simulink model "reference_04_chain_loop_and_merge"  (R2026b)
settings: Solver=FixedStepDiscrete  StartTime=0  StopTime=0.5  FixedStep=0.01  RelTol=1e-10  AbsTol=1e-12
settings Model: Creator=Fasih  LastModifiedBy=Fasih
settings DataIOCC: SaveOutput=off

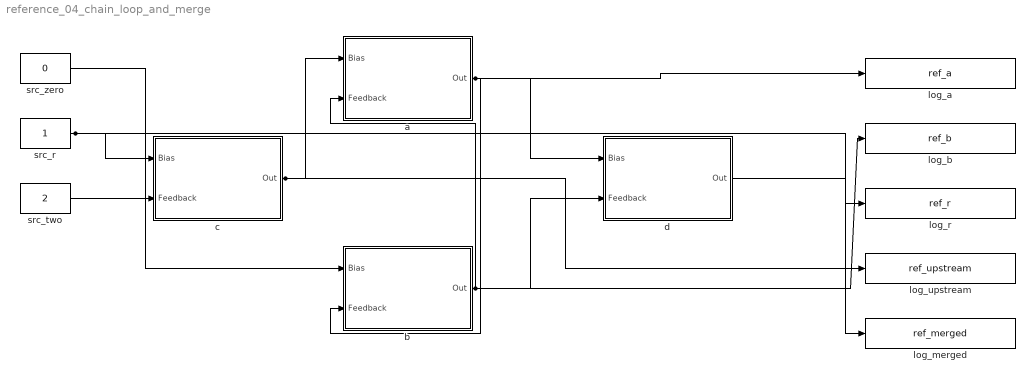
== system reference_04_chain_loop_and_merge ==
  a : Subsystem
  b : Subsystem
  c : Subsystem
  d : Subsystem
  log_a : ToWorkspace  VariableName=ref_a  SaveFormat=Timeseries  SampleTime=0.01
  log_b : ToWorkspace  VariableName=ref_b  SaveFormat=Timeseries  SampleTime=0.01
  log_merged : ToWorkspace  VariableName=ref_merged  SaveFormat=Timeseries  SampleTime=0.01
  log_r : ToWorkspace  VariableName=ref_r  SaveFormat=Timeseries  SampleTime=0.01
  log_upstream : ToWorkspace  VariableName=ref_upstream  SaveFormat=Timeseries  SampleTime=0.01
  src_r : Constant  OutDataTypeStr=double
  src_two : Constant  Value=2  OutDataTypeStr=double
  src_zero : Constant  Value=0  OutDataTypeStr=double
  wires:
  c/1(Out) -> a/1(Bias), log_upstream/1
  src_zero/1 -> b/1(Bias)
  b/1(Out) -> a/2(Feedback), log_b/1, d/2(Feedback)
  a/1(Out) -> b/2(Feedback), log_a/1, d/1(Bias)
  src_r/1 -> log_r/1, c/1(Bias)
  src_two/1 -> c/2(Feedback)
  d/1(Out) -> log_merged/1

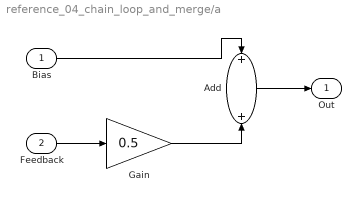
== system reference_04_chain_loop_and_merge/a ==
  Bias : Inport
  Feedback : Inport  Port=2
  Add : Sum
  Gain : Gain  Gain=0.5
  Out : Outport
  wires:
  Bias/1 -> Add/1
  Feedback/1 -> Gain/1
  Gain/1 -> Add/2
  Add/1 -> Out/1

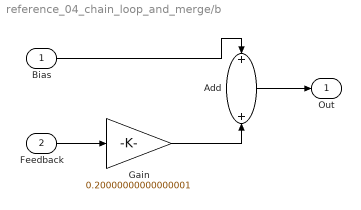
== system reference_04_chain_loop_and_merge/b ==
  Bias : Inport
  Feedback : Inport  Port=2
  Add : Sum
  Gain : Gain  Gain=0.20000000000000001
  Out : Outport
  wires:
  Bias/1 -> Add/1
  Feedback/1 -> Gain/1
  Gain/1 -> Add/2
  Add/1 -> Out/1

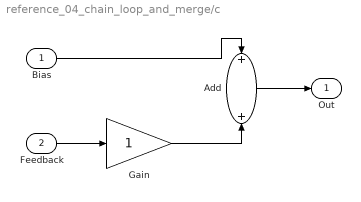
== system reference_04_chain_loop_and_merge/c ==
  Bias : Inport
  Feedback : Inport  Port=2
  Add : Sum
  Gain : Gain
  Out : Outport
  wires:
  Bias/1 -> Add/1
  Feedback/1 -> Gain/1
  Gain/1 -> Add/2
  Add/1 -> Out/1

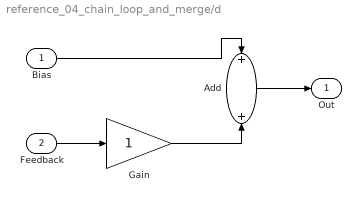
== system reference_04_chain_loop_and_merge/d ==
  Bias : Inport
  Feedback : Inport  Port=2
  Add : Sum
  Gain : Gain
  Out : Outport
  wires:
  Bias/1 -> Add/1
  Feedback/1 -> Gain/1
  Gain/1 -> Add/2
  Add/1 -> Out/1
